simulink model "TLLTD_V2"  (R2025b)
settings: Solver=VariableStepAuto  StartTime=0.0  StopTime=1  RelTol=1e-3
values from neighbouring files (symbols this model uses):
  Centre_of_Gravity = [0.811 0.500 0.280]    [LoadTransferSimulationRevised.m]
  Vehicle_Mass = Sprung_Mass + Front_Unsprung_Mass + Rear_Unsprung_Mass    (= 280.56)    [LoadTransferSimulationRevised.m]
  Wheelbase = 1.56    [LoadTransferSimulationRevised.m]
undefined symbols (not defined in the file or in its folder): Front_Left_Contact_Patch, Front_Right_Contact_Patch, Front_Spring_Stiffness, Rear_Left_Contact_Patch, Rear_Right_Contact_Patch, Rear_Spring_Stiffness
settings Model: Creator=jakub  LastModifiedBy=jakub
settings DataIOCC: SignalLoggingName=loadTransferData

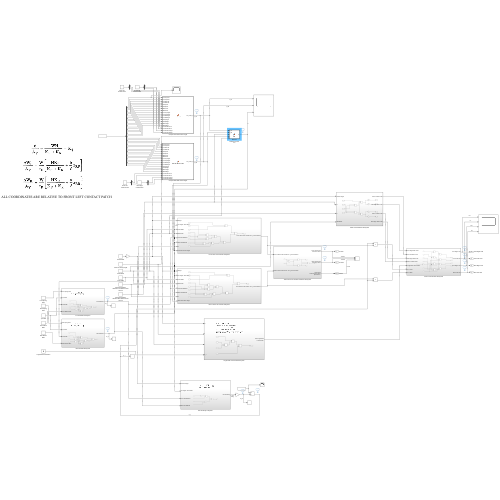
[thumbnail: Simulink's stored preview of the top-level diagram]
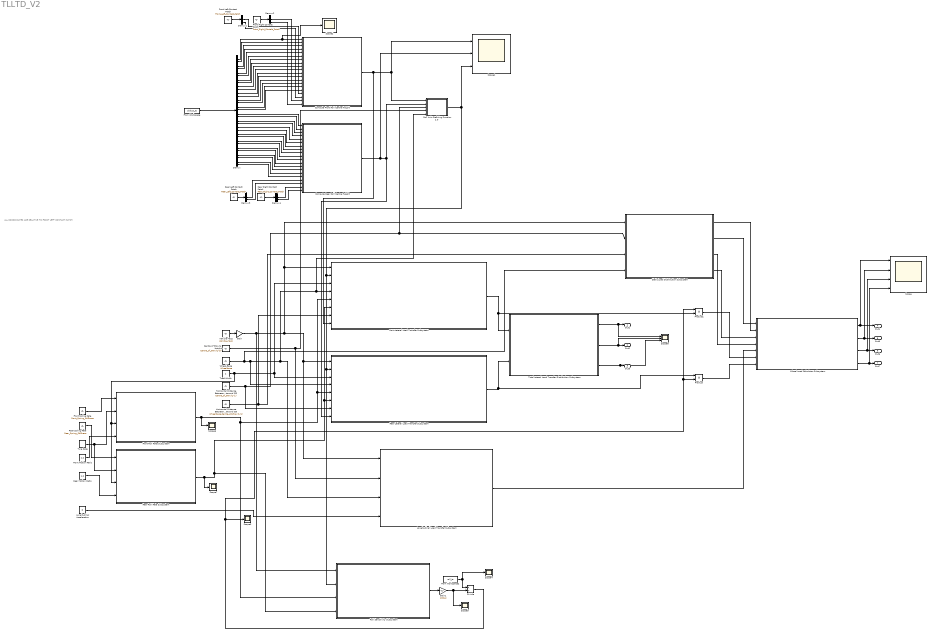
== system TLLTD_V2 ==
  note: ALL COORDINATES ARE RELATIVE TO FRONT LEFT CONTACT PATCH
  Centre of Gravity Height : Constant  Value=Centre_of_Gravity(3)
  Compute Front Roll Centre Height : MATLAB Function  TreatAsAtomicUnit=on
  Compute Rear Roll Centre Height : MATLAB Function  TreatAsAtomicUnit=on
  Demux : Demux  Outputs=48
  Demux{1..4} (4 alike) : Demux  Outputs=3
  Divide : Product  Inputs=*/
  From Workspace : FromWorkspace  VariableName=pickup_ts
  From Workspace2 : FromWorkspace  VariableName=roll_ts
  Front Lateral Load Transfer Subsystem : Subsystem
  Front Left Contact Patch : Constant  Value=Front_Left_Contact_Patch
  Front Motion Ratio : Constant  Value=1.2
  Front Right Contact Patch : Constant  Value=Front_Right_Contact_Patch
  Front Roll Rate Subsystem : Subsystem
  Front Spring Rate : Constant  Value=Front_Spring_Stiffness
  Gain : Gain  Gain=9.81
  Gain1 : Gain  Gain=180/pi
  Horizontal Distance Between Front Wheel Centre and CG : Constant  Value=Centre_of_Gravity(1)
  Horizontal Distance Between Rear Wheel Centre and CG : Constant  Value=Wheelbase-Centre_of_Gravity(1)
  Longitudinal Acceleration : Constant  Value=0
  Longitudinal Load Transfer Subsystem : Subsystem
  Product : Product
  Product1 : Product
  Rear Lateral Load Transfer Subsystem : Subsystem
  Rear Left Contact Patch : Constant  Value=Rear_Left_Contact_Patch
  Rear Motion Ratio : Constant  Value=1.2
  Rear Right Contact Patch : Constant  Value=Rear_Right_Contact_Patch
  Rear Roll Rate Subsystem : Subsystem
  Rear Spring Rate : Constant  Value=Rear_Spring_Stiffness
  Roll Axis Defining Function 2.0 : MATLAB Function  TreatAsAtomicUnit=on
  Roll Sensitivity Subsystem : Subsystem
  Scope : Scope  NumInputPorts=4
      settings: ActiveDisplayYMinimum=-3456.388795993078  ActiveDisplayYMaximum=1756.5748207566396
  Scope1 : Scope  NumInputPorts=3
      settings: ActiveDisplayYMinimum=-4.7305331868134761  ActiveDisplayYMaximum=3.5002061469533192
  Scope{2..7} (6 alike) : Scope
      Scope2 settings: ActiveDisplayYMinimum=-1.2270897028296921  ActiveDisplayYMaximum=1.9019188966833895  DataLoggingVariableName=ScopeData2
      Scope3 settings: ActiveDisplayYMinimum=-45.621537874698639  ActiveDisplayYMaximum=40.415232350486669  DataLoggingVariableName=ScopeData3
      Scope4 settings: ActiveDisplayYMinimum=-13.86030260807604  ActiveDisplayYMaximum=20.17499359623551  DataLoggingVariableName=ScopeData4
      Scope5 settings: ActiveDisplayYMinimum=-0.48971508914464129  ActiveDisplayYMaximum=0.29771268533568446  DataLoggingVariableName=ScopeData5
      Scope6 settings: ActiveDisplayYMinimum=6958.1278970704225  ActiveDisplayYMaximum=46556.759885858381  DataLoggingVariableName=ScopeData6
      Scope7 settings: ActiveDisplayYMinimum=25801.588510961381  ActiveDisplayYMaximum=45801.588510961381  DataLoggingVariableName=ScopeData7
  Scope8 : Scope  NumInputPorts=3
      settings: ActiveDisplayYMinimum=-0.38661831702731586  ActiveDisplayYMaximum=1.5813439493055106  DataLoggingVariableName=ScopeData8
  Static Load Distribution Subsystem : Subsystem
  Total Lateral Load Transfer Distribution Subsystem : Subsystem
  Track-Width : Constant
  Tyre Rate : Constant  Value=125600
  Vehicle Mass : Constant  Value=Vehicle_Mass
  Wheel Load Calculator Subsystem : Subsystem
  Wheel-Base : Constant  Value=Wheelbase
  Out1 : Outport  SignalName=TLLTDF
  Out2 : Outport  Port=2  SignalName=TLLTDR
  Out3 : Outport  Port=3  SignalName=Check
  Out4 : Outport  Port=4  SignalName=Front Right Load
  Out5 : Outport  Port=5  SignalName=Front Left Load
  Out6 : Outport  Port=6  SignalName=Rear Right Load
  Out7 : Outport  Port=7  SignalName=Rear Left Load
  wires:
  Total Lateral Load Transfer Distribution Subsystem/2(Front Lateral Load Transfer Fraction) -> Scope8/2, Out2/1  "TLLTDR"
  Total Lateral Load Transfer Distribution Subsystem/1(Front Load Transfer Fraction) -> Scope8/1, Out1/1  "TLLTDF"
  Total Lateral Load Transfer Distribution Subsystem/3(Check fractions add to unity) -> Scope8/3, Out3/1  "Check"
  Wheel Load Calculator Subsystem/1(Front Right Load) -> Out4/1, Scope/1  "FR"
  Wheel Load Calculator Subsystem/4(Rear Left Load) -> Scope/4, Out7/1  "RL"
  Wheel Load Calculator Subsystem/3(Rear Right Load) -> Out6/1, Scope/3  "RR"
  Wheel Load Calculator Subsystem/2(Front Left Load) -> Out5/1, Scope/2  "FL"
  Track-Width/1 -> Rear Roll Rate Subsystem/3(Trackwidth), Front Roll Rate Subsystem/3(Trackwidth), Front Lateral Load Transfer Subsystem/3(Track Width), Rear Lateral Load Transfer Subsystem/3(Track Width)
  Rear Roll Rate Subsystem/1(Rear Roll Rate) -> Scope7/1, Roll Sensitivity Subsystem/4(Rear Roll Stiffness), Front Lateral Load Transfer Subsystem/6(Rear Roll Stiffness), Rear Lateral Load Transfer Subsystem/6(Rear Roll Stiffness)  "K_R"
  Front Roll Rate Subsystem/1(Front Roll Rate) -> Scope6/1, Roll Sensitivity Subsystem/3(Front Roll Stiffness), Rear Lateral Load Transfer Subsystem/5(Front Roll Stiffness), Front Lateral Load Transfer Subsystem/5(Front Roll Stiffness)  "K_F"
  Longitudinal Acceleration/1 -> Longitudinal Load Transfer Subsystem/4(A_x)
  Horizontal Distance Between Rear Wheel Centre and CG/1 -> Static Load Distribution Subsystem/3(b), Front Lateral Load Transfer Subsystem/7(b)
  Vehicle Mass/1 -> Gain/1
  Gain/1 -> Roll Sensitivity Subsystem/1(Vehicle Weight), Static Load Distribution Subsystem/1(Vehicle Weight), Front Lateral Load Transfer Subsystem/1(Weight), Rear Lateral Load Transfer Subsystem/1(Weight), Longitudinal Load Transfer Subsystem/1(W)
  Longitudinal Load Transfer Subsystem/1(Total Longitudinal Load Transfer) -> Wheel Load Calculator Subsystem/5(Longitudinal Load Transfer)
  Front Lateral Load Transfer Subsystem/1(Front Lateral Load Transfer Per  g of Acceleration) -> Product1/2, Total Lateral Load Transfer Distribution Subsystem/1(Front Lateral Load Transfer Per  g of Acceleration)
  Rear Lateral Load Transfer Subsystem/1(Rear Lateral Load Transfer Per  g of Acceleration) -> Product/1, Total Lateral Load Transfer Distribution Subsystem/2(Rear Lateral Load Transfer Per  g of Acceleration)
  Divide/1 -> Scope3/1, Product1/1, Product/2  "A_y"
  Product1/1 -> Wheel Load Calculator Subsystem/6(TLLT Front)
  Product/1 -> Wheel Load Calculator Subsystem/7(TLLT Rear)
  Static Load Distribution Subsystem/2(Front Right Static Load) -> Wheel Load Calculator Subsystem/1(Front Right Static Load)
  Static Load Distribution Subsystem/1(Front Left Static Load) -> Wheel Load Calculator Subsystem/2(Front Left Static Load)
  Static Load Distribution Subsystem/4(Rear RIght Static Load) -> Wheel Load Calculator Subsystem/3(Rear Right Static Load)
  Static Load Distribution Subsystem/3(Rear Left Static Load) -> Wheel Load Calculator Subsystem/4(Rear Left Static Load)
  Horizontal Distance Between Front Wheel Centre and CG/1 -> Static Load Distribution Subsystem/2(a), Roll Axis Defining Function 2.0/3(a), Rear Lateral Load Transfer Subsystem/7(a)
  Wheel-Base/1 -> Static Load Distribution Subsystem/4(Wheelbase), Rear Lateral Load Transfer Subsystem/4(Wheelbase), Longitudinal Load Transfer Subsystem/3(l), Roll Axis Defining Function 2.0/5(l), Front Lateral Load Transfer Subsystem/4(Wheelbase)
  Compute Rear Roll Centre Height/1(roll_Centre_Z) -> Scope1/2, Rear Lateral Load Transfer Subsystem/8(Rear Roll Centre Height), Roll Axis Defining Function 2.0/2(z_RR)  "z_RR"
  Roll Axis Defining Function 2.0/1(H) -> Roll Sensitivity Subsystem/2(CG Height Above NRA), Rear Lateral Load Transfer Subsystem/2(CG Height Above NRA), Front Lateral Load Transfer Subsystem/2(CG Height Above NRA), Scope1/3  "H"
  Centre of Gravity Height/1 -> Roll Axis Defining Function 2.0/4(h), Longitudinal Load Transfer Subsystem/2(h)
  Compute Front Roll Centre Height/1(roll_Centre_Z) -> Scope1/1, Roll Axis Defining Function 2.0/1(z_RF), Front Lateral Load Transfer Subsystem/8(Front Roll Centre Height)  "z_RF"
  From Workspace/1 -> Demux/1
  Demux/2 -> Scope2/1, Compute Front Roll Centre Height/1(OUTTopYLeft)
  Demux/3 -> Compute Front Roll Centre Height/2(OUTTopZLeft)
  Demux/5 -> Compute Front Roll Centre Height/3(OUTBotYLeft)
  Demux/6 -> Compute Front Roll Centre Height/4(OUTBotZLeft)
  Demux/8 -> Compute Front Roll Centre Height/5(INTopYLeft)
  Demux/9 -> Compute Front Roll Centre Height/6(INTopZLeft)
  Demux/11 -> Compute Front Roll Centre Height/7(INBotYLeft)
  Demux/12 -> Compute Front Roll Centre Height/8(INBotZLeft)
  Demux/14 -> Compute Front Roll Centre Height/9(OUTTopYRight)
  Demux/15 -> Compute Front Roll Centre Height/10(OUTTopZRight)
  Demux/17 -> Compute Front Roll Centre Height/11(OUTBotYRight)
  Demux/18 -> Compute Front Roll Centre Height/12(OUTBotZRight)
  Demux/20 -> Compute Front Roll Centre Height/13(INTopYRight)
  Demux/21 -> Compute Front Roll Centre Height/14(INTopZRight)
  Demux/23 -> Compute Front Roll Centre Height/15(INBotYRight)
  Demux/24 -> Compute Front Roll Centre Height/16(INBotZRight)
  Demux/26 -> Compute Rear Roll Centre Height/1(OUTTopYLeft)
  Demux/27 -> Compute Rear Roll Centre Height/2(OUTTopZLeft)
  Demux/29 -> Compute Rear Roll Centre Height/3(OUTBotYLeft)
  Demux/30 -> Compute Rear Roll Centre Height/4(OUTBotZLeft)
  Demux/32 -> Compute Rear Roll Centre Height/5(INTopYLeft)
  Demux/33 -> Compute Rear Roll Centre Height/6(INTopZLeft)
  Demux/35 -> Compute Rear Roll Centre Height/7(INBotYLeft)
  Demux/36 -> Compute Rear Roll Centre Height/8(INBotZLeft)
  Demux/38 -> Compute Rear Roll Centre Height/9(OUTTopYRight)
  Demux/39 -> Compute Rear Roll Centre Height/10(OUTTopZRight)
  Demux/41 -> Compute Rear Roll Centre Height/11(OUTBotYRight)
  Demux/42 -> Compute Rear Roll Centre Height/12(OUTBotZRight)
  Demux/44 -> Compute Rear Roll Centre Height/13(INTopYRight)
  Demux/45 -> Compute Rear Roll Centre Height/14(INTopZRight)
  Demux/47 -> Compute Rear Roll Centre Height/15(INBotYRight)
  Demux/48 -> Compute Rear Roll Centre Height/16(INBotZRight)
  Front Left Contact Patch/1 -> Demux1/1
  Front Right Contact Patch/1 -> Demux2/1
  Rear Left Contact Patch/1 -> Demux3/1
  Rear Right Contact Patch/1 -> Demux4/1
  Demux1/2 -> Compute Front Roll Centre Height/17(contactPatchYLeft)
  Demux1/3 -> Compute Front Roll Centre Height/18(contactPatchZLeft)
  Demux2/2 -> Compute Front Roll Centre Height/19(contactPatchYRight)
  Demux2/3 -> Compute Front Roll Centre Height/20(contactPatchZRight)
  Demux3/2 -> Compute Rear Roll Centre Height/17(contactPatchYLeft)
  Demux3/3 -> Compute Rear Roll Centre Height/18(contactPatchZLeft)
  Demux4/2 -> Compute Rear Roll Centre Height/19(contactPatchYRight)
  Demux4/3 -> Compute Rear Roll Centre Height/20(contactPatchZRight)
  From Workspace2/1 -> Divide/1, Scope4/1
  Roll Sensitivity Subsystem/1(Roll Sensitivity) -> Gain1/1  "K_phi/ rad/g"
  Gain1/1 -> Scope5/1, Divide/2  "K_phi"
  Front Spring Rate/1 -> Front Roll Rate Subsystem/1(Front Spring Rate)
  Tyre Rate/1 -> Rear Roll Rate Subsystem/2(Tyre Rate), Front Roll Rate Subsystem/2(Tyre Rate)
  Rear Spring Rate/1 -> Rear Roll Rate Subsystem/1(Rear Spring Rate)
  Rear Motion Ratio/1 -> Rear Roll Rate Subsystem/4(Rear Motion Ratio)
  Front Motion Ratio/1 -> Front Roll Rate Subsystem/4(Front Motion Ratio)

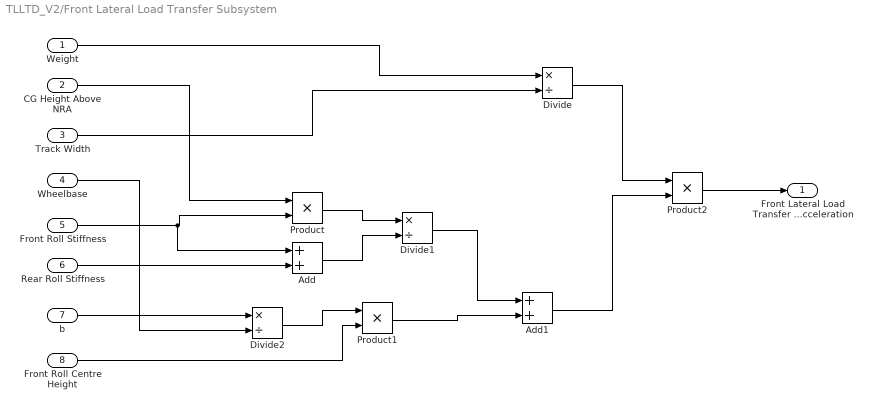
== system TLLTD_V2/Front Lateral Load Transfer Subsystem ==
  Weight : Inport
  CG Height Above NRA : Inport  Port=2
  Track Width : Inport  Port=3
  Wheelbase : Inport  Port=4
  Front Roll Stiffness : Inport  Port=5
  Rear Roll Stiffness : Inport  Port=6
  b : Inport  Port=7
  Front Roll Centre Height : Inport  Port=8
  Add : Sum
  Add1 : Sum
  Divide : Product  Inputs=*/
  Divide1 : Product  Inputs=*/
  Divide2 : Product  Inputs=*/
  Product : Product
  Product1 : Product
  Product2 : Product
  Front Lateral Load Transfer Per  g of Acceleration : Outport
  wires:
  Track Width/1 -> Divide/2
  Weight/1 -> Divide/1
  Front Roll Stiffness/1 -> Add/1, Product/2
  CG Height Above NRA/1 -> Product/1
  Rear Roll Stiffness/1 -> Add/2
  Product/1 -> Divide1/1
  Add/1 -> Divide1/2
  b/1 -> Divide2/1
  Wheelbase/1 -> Divide2/2
  Divide2/1 -> Product1/1
  Front Roll Centre Height/1 -> Product1/2
  Divide1/1 -> Add1/1
  Product1/1 -> Add1/2
  Divide/1 -> Product2/1
  Add1/1 -> Product2/2
  Product2/1 -> Front Lateral Load Transfer Per  g of Acceleration/1

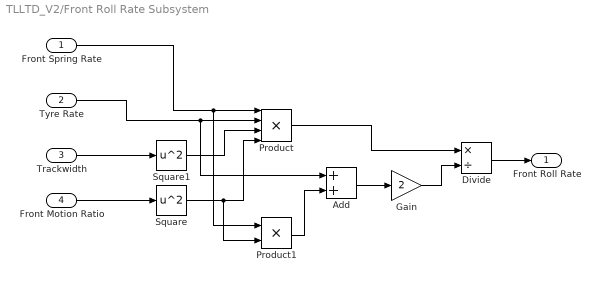
== system TLLTD_V2/Front Roll Rate Subsystem ==
  Front Spring Rate : Inport
  Tyre Rate : Inport  Port=2
  Trackwidth : Inport  Port=3
  Front Motion Ratio : Inport  Port=4
  Add : Sum
  Divide : Product  Inputs=*/
  Gain : Gain  Gain=2
  Product : Product  Inputs=4
  Product1 : Product
  Square : Math  Operator=square
  Square1 : Math  Operator=square
  Front Roll Rate : Outport
  wires:
  Front Motion Ratio/1 -> Square/1
  Trackwidth/1 -> Square1/1
  Square1/1 -> Product/3
  Square/1 -> Product1/2, Product/4
  Front Spring Rate/1 -> Product1/1, Product/1
  Tyre Rate/1 -> Add/1, Product/2
  Product1/1 -> Add/2
  Add/1 -> Gain/1
  Product/1 -> Divide/1
  Gain/1 -> Divide/2
  Divide/1 -> Front Roll Rate/1

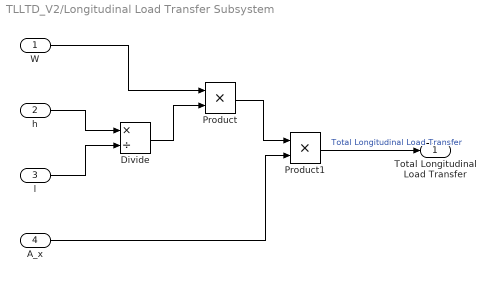
== system TLLTD_V2/Longitudinal Load Transfer Subsystem ==
  W : Inport
  h : Inport  Port=2
  l : Inport  Port=3
  A_x : Inport  Port=4
  Divide : Product  Inputs=*/
  Product : Product
  Product1 : Product
  Total Longitudinal Load Transfer : Outport
  wires:
  Product/1 -> Product1/1
  Product1/1 -> Total Longitudinal Load Transfer/1  "Total Longitudinal Load Transfer"
  Divide/1 -> Product/2
  A_x/1 -> Product1/2
  W/1 -> Product/1
  h/1 -> Divide/1
  l/1 -> Divide/2

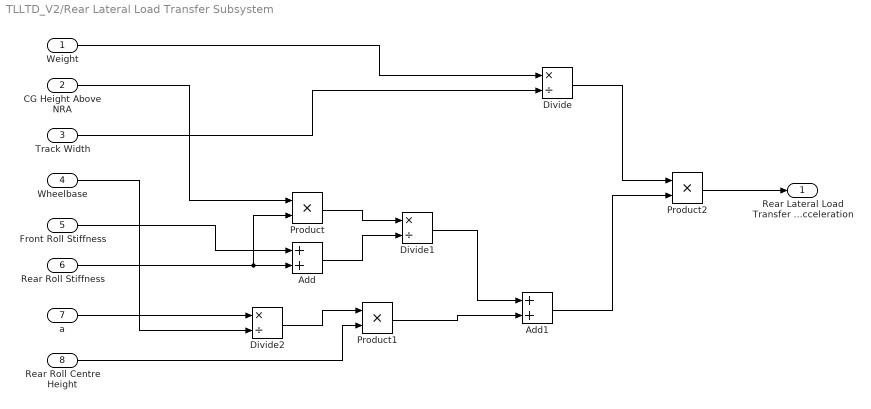
== system TLLTD_V2/Rear Lateral Load Transfer Subsystem ==
  Weight : Inport
  CG Height Above NRA : Inport  Port=2
  Track Width : Inport  Port=3
  Wheelbase : Inport  Port=4
  Front Roll Stiffness : Inport  Port=5
  Rear Roll Stiffness : Inport  Port=6
  a : Inport  Port=7
  Rear Roll Centre Height : Inport  Port=8
  Add : Sum
  Add1 : Sum
  Divide : Product  Inputs=*/
  Divide1 : Product  Inputs=*/
  Divide2 : Product  Inputs=*/
  Product : Product
  Product1 : Product
  Product2 : Product
  Rear Lateral Load Transfer Per  g of Acceleration : Outport
  wires:
  Track Width/1 -> Divide/2
  Weight/1 -> Divide/1
  CG Height Above NRA/1 -> Product/1
  Product/1 -> Divide1/1
  Add/1 -> Divide1/2
  a/1 -> Divide2/1
  Wheelbase/1 -> Divide2/2
  Divide2/1 -> Product1/1
  Rear Roll Centre Height/1 -> Product1/2
  Divide1/1 -> Add1/1
  Product1/1 -> Add1/2
  Divide/1 -> Product2/1
  Add1/1 -> Product2/2
  Product2/1 -> Rear Lateral Load Transfer Per  g of Acceleration/1
  Rear Roll Stiffness/1 -> Product/2, Add/2
  Front Roll Stiffness/1 -> Add/1

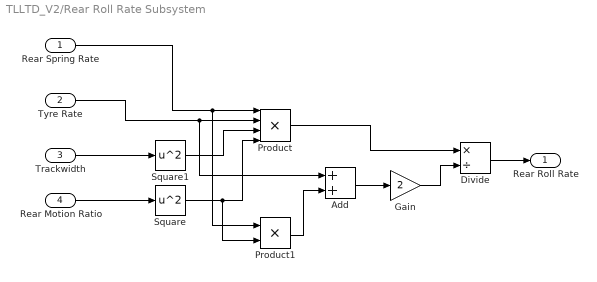
== system TLLTD_V2/Rear Roll Rate Subsystem ==
  Rear Spring Rate : Inport
  Tyre Rate : Inport  Port=2
  Trackwidth : Inport  Port=3
  Rear Motion Ratio : Inport  Port=4
  Add : Sum
  Divide : Product  Inputs=*/
  Gain : Gain  Gain=2
  Product : Product  Inputs=4
  Product1 : Product
  Square : Math  Operator=square
  Square1 : Math  Operator=square
  Rear Roll Rate : Outport
  wires:
  Rear Motion Ratio/1 -> Square/1
  Trackwidth/1 -> Square1/1
  Square1/1 -> Product/3
  Square/1 -> Product1/2, Product/4
  Rear Spring Rate/1 -> Product1/1, Product/1
  Tyre Rate/1 -> Add/1, Product/2
  Product1/1 -> Add/2
  Add/1 -> Gain/1
  Product/1 -> Divide/1
  Gain/1 -> Divide/2
  Divide/1 -> Rear Roll Rate/1

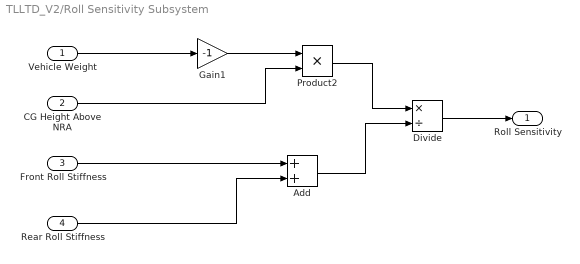
== system TLLTD_V2/Roll Sensitivity Subsystem ==
  Vehicle Weight : Inport
  CG Height Above NRA : Inport  Port=2
  Front Roll Stiffness : Inport  Port=3
  Rear Roll Stiffness : Inport  Port=4
  Add : Sum
  Divide : Product  Inputs=*/
  Gain1 : Gain  Gain=-1
  Product2 : Product
  Roll Sensitivity : Outport
  wires:
  Gain1/1 -> Product2/1
  Product2/1 -> Divide/1
  Divide/1 -> Roll Sensitivity/1
  Add/1 -> Divide/2
  Vehicle Weight/1 -> Gain1/1
  CG Height Above NRA/1 -> Product2/2
  Front Roll Stiffness/1 -> Add/1
  Rear Roll Stiffness/1 -> Add/2

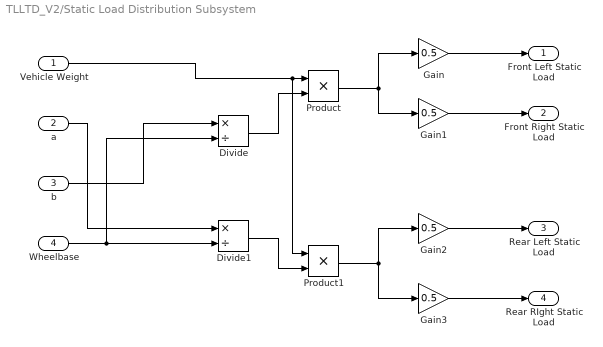
== system TLLTD_V2/Static Load Distribution Subsystem ==
  Vehicle Weight : Inport
  a : Inport  Port=2
  b : Inport  Port=3
  Wheelbase : Inport  Port=4
  Divide : Product  Inputs=*/
  Divide1 : Product  Inputs=*/
  Gain{,1..3} (4 alike) : Gain  Gain=0.5
  Product : Product
  Product1 : Product
  Front Left Static Load : Outport
  Front Right Static Load : Outport  Port=2
  Rear Left Static Load : Outport  Port=3
  Rear RIght Static Load : Outport  Port=4
  wires:
  b/1 -> Divide/1
  Wheelbase/1 -> Divide/2, Divide1/2
  Vehicle Weight/1 -> Product1/1, Product/1
  Divide/1 -> Product/2
  Product/1 -> Gain1/1, Gain/1
  Gain/1 -> Front Left Static Load/1
  Gain1/1 -> Front Right Static Load/1
  a/1 -> Divide1/1
  Divide1/1 -> Product1/2
  Gain3/1 -> Rear RIght Static Load/1
  Gain2/1 -> Rear Left Static Load/1
  Product1/1 -> Gain2/1, Gain3/1

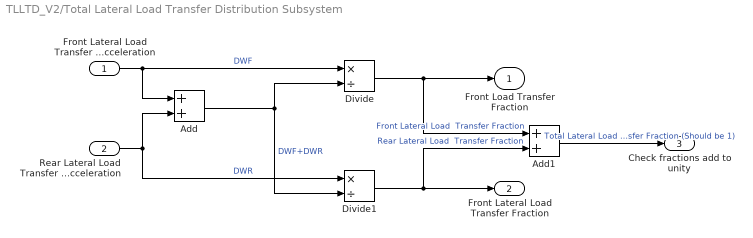
== system TLLTD_V2/Total Lateral Load Transfer Distribution Subsystem ==
  Front Lateral Load Transfer Per  g of Acceleration : Inport
  Rear Lateral Load Transfer Per  g of Acceleration : Inport  Port=2
  Add : Sum
  Add1 : Sum
  Divide : Product  Inputs=*/
  Divide1 : Product  Inputs=*/
  Front Load Transfer Fraction : Outport
  Front Lateral Load Transfer Fraction : Outport  Port=2
  Check fractions add to unity : Outport  Port=3
  wires:
  Add1/1 -> Check fractions add to unity/1  "Total Lateral Load Transfer Fraction (Should be 1)"
  Divide1/1 -> Front Lateral Load Transfer Fraction/1, Add1/2  "Rear Lateral Load  Transfer Fraction"
  Add/1 -> Divide1/2, Divide/2  "DWF+DWR"
  Divide/1 -> Front Load Transfer Fraction/1, Add1/1  "Front Lateral Load  Transfer Fraction"
  Front Lateral Load Transfer Per  g of Acceleration/1 -> Add/1, Divide/1  "DWF"
  Rear Lateral Load Transfer Per  g of Acceleration/1 -> Divide1/1, Add/2  "DWR"

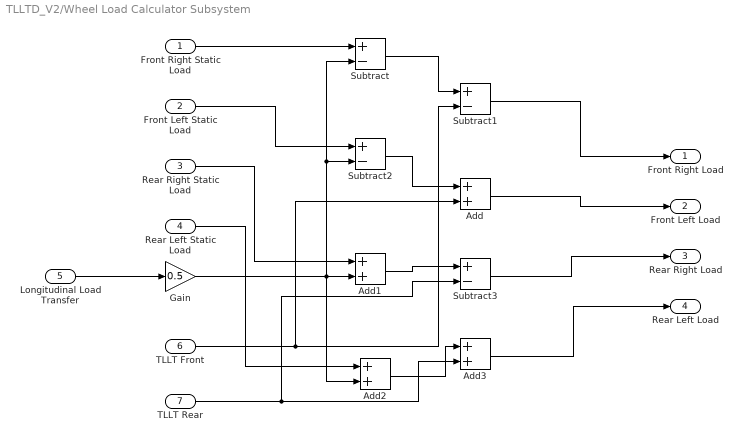
== system TLLTD_V2/Wheel Load Calculator Subsystem ==
  Front Right Static Load : Inport
  Front Left Static Load : Inport  Port=2
  Rear Right Static Load : Inport  Port=3
  Rear Left Static Load : Inport  Port=4
  Longitudinal Load Transfer : Inport  Port=5
  TLLT Front : Inport  Port=6
  TLLT Rear : Inport  Port=7
  Add{,1..3} (4 alike) : Sum
  Gain : Gain  Gain=0.5
  Subtract{,1..3} (4 alike) : Sum  Inputs=+-
  Front Right Load : Outport
  Front Left Load : Outport  Port=2
  Rear Right Load : Outport  Port=3
  Rear Left Load : Outport  Port=4
  wires:
  Front Right Static Load/1 -> Subtract/1
  Longitudinal Load Transfer/1 -> Gain/1
  TLLT Front/1 -> Add/2, Subtract1/2
  Subtract/1 -> Subtract1/1
  Subtract1/1 -> Front Right Load/1
  Front Left Static Load/1 -> Subtract2/1
  Subtract2/1 -> Add/1
  TLLT Rear/1 -> Add3/2, Subtract3/2
  Add/1 -> Front Left Load/1
  Rear Right Static Load/1 -> Add1/1
  Add1/1 -> Subtract3/1
  Subtract3/1 -> Rear Right Load/1
  Rear Left Static Load/1 -> Add2/1
  Add2/1 -> Add3/1
  Add3/1 -> Rear Left Load/1
  Gain/1 -> Add2/2, Subtract2/2, Subtract/2, Add1/2

== matlab function TLLTD_V2/Compute Front Roll Centre Height ==
  data: OUTTopYLeft input; roll_Centre_Z output; OUTTopZLeft input; OUTBotYLeft input; OUTBotZLeft input; INTopYLeft input; INTopZLeft input; INBotYLeft input; INBotZLeft input; OUTTopYRight input; OUTTopZRight input; OUTBotYRight input; OUTBotZRight input; INTopYRight input; INTopZRight input; INBotYRight input; INBotZRight input; contactPatchYLeft input; contactPatchZLeft input; contactPatchYRight input; contactPatchZRight input
function roll_Centre_Z = compute_Roll_Centre(OUTTopYLeft,OUTTopZLeft,OUTBotYLeft,OUTBotZLeft, ...
    INTopYLeft,INTopZLeft,INBotYLeft,INBotZLeft,OUTTopYRight,OUTTopZRight,OUTBotYRight,OUTBotZRight, ...
    INTopYRight,INTopZRight,INBotYRight,INBotZRight,contactPatchYLeft,contactPatchZLeft,contactPatchYRight, ...
    contactPatchZRight)

% Input coordinates should be relative to an origin at the FRONT LEFT TYRE
% CONTACT PATCH

% If coordinates area relative to vehicle centre of gravity, coordinate
%transforms must first be done


%%%%%%%%%%%%%%%%%%%%%%%%%% LEFT INSTANT CENTRE %%%%%%%%%%%%%%%%%%%%%%%%%%%%

OUTTopLeft = [OUTTopYLeft OUTTopZLeft]
OUTBotLeft = [OUTBotYLeft OUTBotZLeft]

INTopLeft = [INTopYLeft INTopZLeft]
INBotLeft = [INBotYLeft INBotZLeft]

gradient_Top_Left = (INTopLeft(2) - OUTTopLeft(2))/(INTopLeft(1)-OUTTopLeft(1))
gradient_Bot_Left = (INBotLeft(2) - OUTBotLeft(2))/(INBotLeft(1)-OUTBotLeft(1))

inst_Centre_Y_Left = (gradient_Top_Left*OUTTopLeft(1)-gradient_Bot_Left*OUTBotLeft(1)+OUTBotLeft(2)- ...
                 OUTTopLeft(2))/(gradient_Top_Left-gradient_Bot_Left)

inst_Centre_Z_Left = gradient_Top_Left*(inst_Centre_Y_Left-OUTTopLeft(1))+OUTTopLeft(2)

%%%%%%%%%%%%%%%%%%%%%%%%%%%%%%%%%%%%%%%%%%%%%%%%%%%%%%%%%%%%%%%%%%%%%%%%%%%

%%%%%%%%%%%%%%%%%%%%%%%%%% RIGHT INSTANT CENTRE %%%%%%%%%%%%%%%%%%%%%%%%%%%

OUTTopRight = [OUTTopYRight OUTTopZRight]
OUTBotRight = [OUTBotYRight OUTBotZRight]

INTopRight = [INTopYRight INTopZRight]
INBotRight = [INBotYRight INBotZRight]

gradient_Top_Right = (INTopRight(2) - OUTTopRight(2))/(INTopRight(1)-OUTTopRight(1))
gradient_Bot_Right = (INBotRight(2) - OUTBotRight(2))/(INBotRight(1)-OUTBotRight(1))

inst_Centre_Y_Right = (gradient_Top_Right*OUTTopRight(1)-gradient_Bot_Right*OUTBotRight(1)+OUTBotRight(2)- ...
                 OUTTopRight(2))/(gradient_Top_Right-gradient_Bot_Right)

inst_Centre_Z_Right = gradient_Top_Right*(inst_Centre_Y_Right-OUTTopRight(1))+OUTTopRight(2)

%%%%%%%%%%%%%%%%%%%%%%%%%%%%%%%%%%%%%%%%%%%%%%%%%%%%%%%%%%%%%%%%%%%%%%%%%%%

%%%%%%%%%%%%%%%%%%%%%%%%%% ROLL CENTRE CALCULATION %%%%%%%%%%%%%%%%%%%%%%%%

inst_Centre_Right = [inst_Centre_Y_Right inst_Centre_Z_Right]
inst_Centre_Left = [inst_Centre_Y_Left inst_Centre_Z_Left]

contact_Patch_Left = [contactPatchYLeft contactPatchZLeft]
contact_Patch_Right = [contactPatchYRight contactPatchZRight]



slope_CP_to_IC_Left = (inst_Centre_Left(2) - contact_Patch_Left(2))/(inst_Centre_Left(1)-contact_Patch_Left(1))
slope_CP_to_IC_Right = (inst_Centre_Right(2) - contact_Patch_Right(2))/(inst_Centre_Right(1)-contact_Patch_Right(1))

roll_Centre_Y = (slope_CP_to_IC_Right*inst_Centre_Right(1)-slope_CP_to_IC_Left*inst_Centre_Left(1)+inst_Centre_Left(2)- ...
                 inst_Centre_Right(2))/(slope_CP_to_IC_Right-slope_CP_to_IC_Left)

roll_Centre_Z = slope_CP_to_IC_Right*(roll_Centre_Y-inst_Centre_Right(1)) + inst_Centre_Right(2)

%%%%%%%%%%%%%%%%%%%%%%%%%%%%%%%%%%%%%%%%%%%%%%%%%%%%%%%%%%%%%%%%%%%%%%%%%%%

end

== matlab function TLLTD_V2/Compute Rear Roll Centre Height ==
  data: OUTTopYLeft input; roll_Centre_Z output; OUTTopZLeft input; OUTBotYLeft input; OUTBotZLeft input; INTopYLeft input; INTopZLeft input; INBotYLeft input; INBotZLeft input; OUTTopYRight input; OUTTopZRight input; OUTBotYRight input; OUTBotZRight input; INTopYRight input; INTopZRight input; INBotYRight input; INBotZRight input; contactPatchYLeft input; contactPatchZLeft input; contactPatchYRight input; contactPatchZRight input
function roll_Centre_Z = compute_Roll_Centre(OUTTopYLeft,OUTTopZLeft,OUTBotYLeft,OUTBotZLeft, ...
    INTopYLeft,INTopZLeft,INBotYLeft,INBotZLeft,OUTTopYRight,OUTTopZRight,OUTBotYRight,OUTBotZRight, ...
    INTopYRight,INTopZRight,INBotYRight,INBotZRight,contactPatchYLeft,contactPatchZLeft,contactPatchYRight, ...
    contactPatchZRight)

% Input coordinates should be relative to an origin at the FRONT LEFT TYRE
% CONTACT PATCH

% If coordinates area relative to vehicle centre of gravity, coordinate
%transforms must first be done


%%%%%%%%%%%%%%%%%%%%%%%%%% LEFT INSTANT CENTRE %%%%%%%%%%%%%%%%%%%%%%%%%%%%

OUTTopLeft = [OUTTopYLeft OUTTopZLeft]
OUTBotLeft = [OUTBotYLeft OUTBotZLeft]

INTopLeft = [INTopYLeft INTopZLeft]
INBotLeft = [INBotYLeft INBotZLeft]

gradient_Top_Left = (INTopLeft(2) - OUTTopLeft(2))/(INTopLeft(1)-OUTTopLeft(1))
gradient_Bot_Left = (INBotLeft(2) - OUTBotLeft(2))/(INBotLeft(1)-OUTBotLeft(1))

inst_Centre_Y_Left = (gradient_Top_Left*OUTTopLeft(1)-gradient_Bot_Left*OUTBotLeft(1)+OUTBotLeft(2)- ...
                 OUTTopLeft(2))/(gradient_Top_Left-gradient_Bot_Left)

inst_Centre_Z_Left = gradient_Top_Left*(inst_Centre_Y_Left-OUTTopLeft(1))+OUTTopLeft(2)

%%%%%%%%%%%%%%%%%%%%%%%%%%%%%%%%%%%%%%%%%%%%%%%%%%%%%%%%%%%%%%%%%%%%%%%%%%%

%%%%%%%%%%%%%%%%%%%%%%%%%% RIGHT INSTANT CENTRE %%%%%%%%%%%%%%%%%%%%%%%%%%%

OUTTopRight = [OUTTopYRight OUTTopZRight]
OUTBotRight = [OUTBotYRight OUTBotZRight]

INTopRight = [INTopYRight INTopZRight]
INBotRight = [INBotYRight INBotZRight]

gradient_Top_Right = (INTopRight(2) - OUTTopRight(2))/(INTopRight(1)-OUTTopRight(1))
gradient_Bot_Right = (INBotRight(2) - OUTBotRight(2))/(INBotRight(1)-OUTBotRight(1))

inst_Centre_Y_Right = (gradient_Top_Right*OUTTopRight(1)-gradient_Bot_Right*OUTBotRight(1)+OUTBotRight(2)- ...
                 OUTTopRight(2))/(gradient_Top_Right-gradient_Bot_Right)

inst_Centre_Z_Right = gradient_Top_Right*(inst_Centre_Y_Right-OUTTopRight(1))+OUTTopRight(2)

%%%%%%%%%%%%%%%%%%%%%%%%%%%%%%%%%%%%%%%%%%%%%%%%%%%%%%%%%%%%%%%%%%%%%%%%%%%

%%%%%%%%%%%%%%%%%%%%%%%%%% ROLL CENTRE CALCULATION %%%%%%%%%%%%%%%%%%%%%%%%

inst_Centre_Right = [inst_Centre_Y_Right inst_Centre_Z_Right]
inst_Centre_Left = [inst_Centre_Y_Left inst_Centre_Z_Left]

contact_Patch_Left = [contactPatchYLeft contactPatchZLeft]
contact_Patch_Right = [contactPatchYRight contactPatchZRight]



slope_CP_to_IC_Left = (inst_Centre_Left(2) - contact_Patch_Left(2))/(inst_Centre_Left(1)-contact_Patch_Left(1))
slope_CP_to_IC_Right = (inst_Centre_Right(2) - contact_Patch_Right(2))/(inst_Centre_Right(1)-contact_Patch_Right(1))

roll_Centre_Y = (slope_CP_to_IC_Right*inst_Centre_Right(1)-slope_CP_to_IC_Left*inst_Centre_Left(1)+inst_Centre_Left(2)- ...
                 inst_Centre_Right(2))/(slope_CP_to_IC_Right-slope_CP_to_IC_Left)

roll_Centre_Z = slope_CP_to_IC_Right*(roll_Centre_Y-inst_Centre_Right(1)) + inst_Centre_Right(2)

%%%%%%%%%%%%%%%%%%%%%%%%%%%%%%%%%%%%%%%%%%%%%%%%%%%%%%%%%%%%%%%%%%%%%%%%%%%

end

== matlab function TLLTD_V2/Roll Axis Defining Function 2.0 ==
  data: z_RF input; H output; z_RR input; a input; h input; l input
function H = fcn(z_RF, z_RR, a, h, l)

% z_RF = Front roll centre height
% z_RR = Rear roll centre height

frontRoll = [0 z_RF]
rearRoll = [l z_RR]
CG = [a h]

NRA = rearRoll - frontRoll
NRA_below_CG = frontRoll + a/l*(NRA)
H = norm(CG-NRA_below_CG)

end
